simulink model "S12_hellcat_2022_stock_v12_texture_candidate"  (R2026a)
settings: Solver=FixedStepDiscrete  StopTime=89.98  FixedStep=0.02
undefined symbols (not defined in the file): s12_v12_model_source_step, s12_v12_model_stereo_renderer_step, s12_v12_model_vehicle_cycle_step
settings Model: Creator=Jovi  LastModifiedBy=Jovi

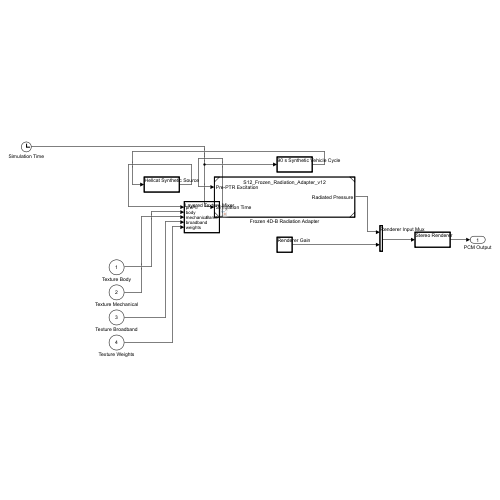
[thumbnail: Simulink's stored preview of the top-level diagram]
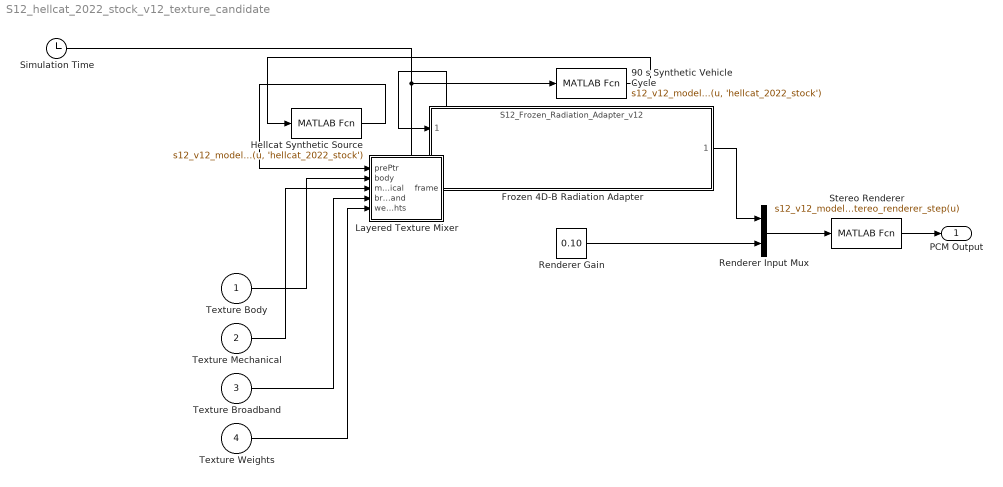
== system S12_hellcat_2022_stock_v12_texture_candidate ==
  Texture Body : Inport  OutDataTypeStr=double  PortDimensions=[960 1]  SampleTime=0.02  Interpolate=off
  Texture Mechanical : Inport  Port=2  OutDataTypeStr=double  PortDimensions=[960 1]  SampleTime=0.02  Interpolate=off
  Texture Broadband : Inport  Port=3  OutDataTypeStr=double  PortDimensions=[960 1]  SampleTime=0.02  Interpolate=off
  Texture Weights : Inport  Port=4  OutDataTypeStr=double  PortDimensions=[1 3]  SampleTime=0.02  Interpolate=off
  90 s Synthetic Vehicle Cycle : MATLABFcn  MATLABFcn=s12_v12_model_vehicle_cycle_step(u, 'hellcat_2022_stock')  OutputDimensions=[9 1]  Output1D=off
  Frozen 4D-B Radiation Adapter : ModelReference  ModelNameDialog=S12_Frozen_Radiation_Adapter_v12  SimulationMode=Normal  ModelReferenceVersion=1.1
  Hellcat Synthetic Source : MATLABFcn  MATLABFcn=s12_v12_model_source_step(u, 'hellcat_2022_stock')  OutputDimensions=[960 1]  Output1D=off
  Layered Texture Mixer : MATLAB Function  TreatAsAtomicUnit=on
  Renderer Gain : Constant  Value=0.10
  Renderer Input Mux : Mux  Inputs=2
  Simulation Time : Clock
  Stereo Renderer : MATLABFcn  MATLABFcn=s12_v12_model_stereo_renderer_step(u)  OutputDimensions=[960 2]  Output1D=off
  PCM Output : Outport  PortDimensions=[960 2]
  wires:
  90 s Synthetic Vehicle Cycle/1 -> Hellcat Synthetic Source/1
  Simulation Time/1 -> Frozen 4D-B Radiation Adapter/2, 90 s Synthetic Vehicle Cycle/1
  Frozen 4D-B Radiation Adapter/1 -> Renderer Input Mux/1
  Renderer Gain/1 -> Renderer Input Mux/2
  Renderer Input Mux/1 -> Stereo Renderer/1
  Stereo Renderer/1 -> PCM Output/1
  Hellcat Synthetic Source/1 -> Layered Texture Mixer/1(prePtr)
  Texture Body/1 -> Layered Texture Mixer/2(body)
  Texture Mechanical/1 -> Layered Texture Mixer/3(mechanical)
  Texture Broadband/1 -> Layered Texture Mixer/4(broadband)
  Texture Weights/1 -> Layered Texture Mixer/5(weights)
  Layered Texture Mixer/1(frame) -> Frozen 4D-B Radiation Adapter/1

== matlab function S12_hellcat_2022_stock_v12_texture_candidate/Layered Texture Mixer ==
  data: prePtr input double size=[960 1]; frame output double size=[960 1]; body input double size=[960 1]; mechanical input double size=[960 1]; broadband input double size=[960 1]; weights input double size=[1 3]
function frame = fcn(prePtr, body, mechanical, broadband, weights)
frame = s12_v12_model_texture_layers_step(prePtr,body,mechanical,broadband,weights);
end
